simulink model "PID"  (R2025b)
settings: Solver=FixedStepAuto  StartTime=0.0  StopTime=10.0  FixedStep=0.01  RelTol=1e-3
undefined symbols (not defined in the file): b, c, g, I, kb, kt, l, M, m, r, Rm
libraries: vrlib x3, slpidlib x2
settings Model: Creator=jitendra  LastModifiedBy=joelalfaro
settings SolverCC: AlgebraicLoopSolver=TrustRegion
settings DataIOCC: ExternalInput=getinputstruct(op_trim1)  InitialState=getstatestruct(op_trim1)  ReturnWorkspaceOutputs=off
settings DebuggingCC: UnconnectedInputMsg=warning  UnconnectedOutputMsg=warning  UnconnectedLineMsg=warning  ArithmeticOperatorsInVariantConditions=warning
settings ModelReferenceCC: EnableRefExpFcnMdlSchedulingChecks=on
settings SFSimCC: SimUseLocalCustomCode=off  CustomCodeUndefinedFunction=UseInterfaceOnly
settings RTWCC: RTWUseLocalCustomCode=off  GPUComputeCapability=3.5

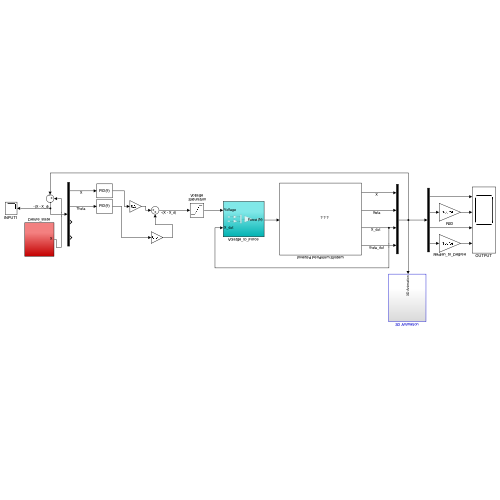
[thumbnail: Simulink's stored preview of the top-level diagram]
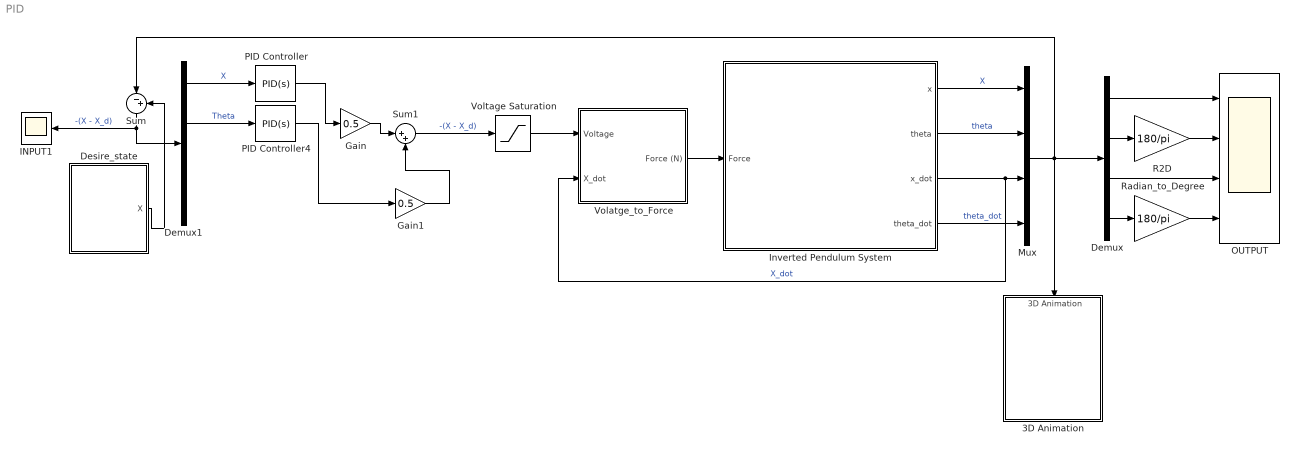
== system PID ==
  3D Animation : Subsystem
      settings: PortSchema="{\"entries\":[{\"content\":{\"sides\":[{\"content\":{},\"type\":\"ConnectorPlacement.EquallySpacedRectSide\",\"uuid\":\"e4203b7e-781e-4354-bf67-6c487e3884b6\"},{\"content\":{\"side\":\"RIGHT\"},\"type\":\"ConnectorPlacement.EquallySpacedRectSide\",\"uuid\":\"7bd3bb4e-855c-4795-9350-7e2ed6adbf10\"},{\"content\":{\"connectorIds\":[\"In1\"],\"side\":\"TOP\"},\"type\":\"ConnectorPlacement.EquallySpacedRectSide\",\"uuid\":\"c2ae83d0-35fa-4ceb-879c-e55f231126ee\"}]},\"type\":\"ConnectorPlacement.EquallySpacedConnector\",\"uuid\":\"fb632b4d-2504-45df-9ed9-db3d660227bd\"}],\"packageUris\":[\"http://schema.mathworks.com/mf0/Connector/R2020b\"],\"version\":\"1.0\"}"
  Demux : Demux
  Demux1 : Demux
  Desire_state : Subsystem
  Gain : Gain  Gain=0.5
  Gain1 : Gain  Gain=0.5
  INPUT1 : Scope
      settings: ActiveDisplayYMinimum=-15  ActiveDisplayYMaximum=15
  Inverted Pendulum System : Subsystem
      mask Display: image('ip_model.png');
  Mux : Mux
  OUTPUT : Scope  NumInputPorts=4
      settings: ActiveDisplayString=4  ActiveDisplayYMinimum=-139.60429875287392  ActiveDisplayYMaximum=335.60525389864625  YLabel=\theta dot (deg/sec)
  PID Controller : slpidlib/PID Controller  Controller=PID  Form=Parallel  TimeDomain=Continuous-time  UseExternalTs=off  SampleTime=-1  IntegratorMethod=Forward Euler  FilterMethod=Forward Euler  ControllerParametersSource=internal  P=-58.450  I=-25.45  UseKiTs=off  D=-5.57  UseExternalDerivativeSource=off  N=100  UseFilter=on  TunerSelectOption=Transfer Function Based (PID Tuner App)  InitialConditionSource=internal  InitialConditionForIntegrator=0  InitialConditionForFilter=0  DifferentiatorICPrevScaledInput=0  ExternalReset=none  TrackingMode=off  Kt=1  LimitOutput=off  SatLimitsSource=internal  UpperSaturationLimit=inf  LowerSaturationLimit=-inf  LinearizeAsGain=on  AntiWindupMode=none  Kb=1  LimitIntegrator=off  UpperIntegratorSaturationLimit=inf  LowerIntegratorSaturationLimit=-inf  POutMin=[]  POutMax=[]  IOutMin=[]  IOutMax=[]  DOutMin=[]  DOutMax=[]  NOutMin=[]  NOutMax=[]  SumOutMin=[]  SumOutMax=[]  SaturationOutMin=[]  SaturationOutMax=[]  PParamMin=[]  PParamMax=[]  IParamMin=[]  IParamMax=[]  DParamMin=[]  DParamMax=[]  NParamMin=[]  NParamMax=[]  KbParamMin=[]  KbParamMax=[]  KtParamMin=[]  KtParamMax=[]  KbOutMin=[]  KbOutMax=[]  KtOutMin=[]  KtOutMax=[]  IntegratorOutMin=[]  IntegratorOutMax=[]  FilterOutMin=[]  FilterOutMax=[]  SumI1OutMin=[]  SumI1OutMax=[]  SumI2OutMin=[]  SumI2OutMax=[]  SumI3OutMin=[]  SumI3OutMax=[]  SumI4OutMin=[]  SumI4OutMax=[]  SumDOutMin=[]  SumDOutMax=[]  DifferentiatorOutMin=[]  DifferentiatorOutMax=[]  FilterDiffOutCoefMin=[]  FilterDiffOutCoefMax=[]  ReciprocalOutMin=[]  ReciprocalOutMax=[]  SumDenOutMin=[]  SumDenOutMax=[]  SumNumOutMin=[]  SumNumOutMax=[]  DivideOutMin=[]  DivideOutMax=[]  UdiffTsProdOutMin=[]  UdiffTsProdOutMax=[]  NTsProdOutMin=[]  NTsProdOutMax=[]  UintegralTsProdOutMin=[]  UintegralTsProdOutMax=[]  UngainTsProdOutMin=[]  UngainTsProdOutMax=[]  ClampingZeroOutDataTypeStr=Inherit: Inherit via back propagation  ClampingZeroOutMin=[]  ClampingZeroOutMax=[]  FilterDenConstantOutDataTypeStr=Inherit: Inherit via back propagation  FilterDenConstantOutMin=[]  FilterDenConstantOutMax=[]  PCopyOutDataTypeStr=Inherit: Inherit via back propagation  PCopyOutMin=[]  PCopyOutMax=[]  NCopyOutDataTypeStr=Inherit: Inherit via back propagation  NCopyOutMin=[]  NCopyOutMax=[]  IntegratorContinuousStateAttributes=''  IntegratorStateMustResolveToSignalObject=off  IntegratorRTWStateStorageClass=Auto  FilterContinuousStateAttributes=''  FilterStateMustResolveToSignalObject=off  FilterRTWStateStorageClass=Auto  ParallelPVariant=InternalParameters  IdealPVariant=Disabled  IVariant=InternalParameters  DVariant=InternalParameters  IntegratorVariant=Continuous  SatVariant=Disabled  AWVariant=Passthrough  PCopyVariant=Disabled  TRVariant=Disabled  FdbkBlocksVariant=Forward  IdealPFdbkVariant=Disabled  SatFdbkVariant=Disabled  DerivativeFilterVariant=ContFilter  NVariant=InternalParameters  NCopyVariant=Disabled  FilterICVariant=InternalICsFilter  IntegratorICVariant=InternalICs  ExternalResetVariant=Disabled  TRSumVariant=Passthrough  SumFdbkVariant=Disabled  SumVariant=Sum_PID  TsampFilterVariant=InternalTs  TsampNgainVariant=Passthrough  TsampIntegralVariant=Disabled_SignalSpec  ExternalSaturationOutDataTypeStr=Inherit: Same as second input  DerivativeSourceVariant=ErrorSignal  PreIntVariant=InternalPreInt
  PID Controller4 : slpidlib/PID Controller  Controller=PID  Form=Parallel  TimeDomain=Continuous-time  UseExternalTs=off  SampleTime=-1  IntegratorMethod=Forward Euler  FilterMethod=Forward Euler  ControllerParametersSource=internal  P=120.5493  I=775.1235  UseKiTs=off  D=5.2021  UseExternalDerivativeSource=off  N=100  UseFilter=on  TunerSelectOption=Transfer Function Based (PID Tuner App)  InitialConditionSource=internal  InitialConditionForIntegrator=0  InitialConditionForFilter=0  DifferentiatorICPrevScaledInput=0  ExternalReset=none  TrackingMode=off  Kt=1  LimitOutput=off  SatLimitsSource=internal  UpperSaturationLimit=inf  LowerSaturationLimit=-inf  LinearizeAsGain=on  AntiWindupMode=none  Kb=1  LimitIntegrator=off  UpperIntegratorSaturationLimit=inf  LowerIntegratorSaturationLimit=-inf  POutMin=[]  POutMax=[]  IOutMin=[]  IOutMax=[]  DOutMin=[]  DOutMax=[]  NOutMin=[]  NOutMax=[]  SumOutMin=[]  SumOutMax=[]  SaturationOutMin=[]  SaturationOutMax=[]  PParamMin=[]  PParamMax=[]  IParamMin=[]  IParamMax=[]  DParamMin=[]  DParamMax=[]  NParamMin=[]  NParamMax=[]  KbParamMin=[]  KbParamMax=[]  KtParamMin=[]  KtParamMax=[]  KbOutMin=[]  KbOutMax=[]  KtOutMin=[]  KtOutMax=[]  IntegratorOutMin=[]  IntegratorOutMax=[]  FilterOutMin=[]  FilterOutMax=[]  SumI1OutMin=[]  SumI1OutMax=[]  SumI2OutMin=[]  SumI2OutMax=[]  SumI3OutMin=[]  SumI3OutMax=[]  SumI4OutMin=[]  SumI4OutMax=[]  SumDOutMin=[]  SumDOutMax=[]  DifferentiatorOutMin=[]  DifferentiatorOutMax=[]  FilterDiffOutCoefMin=[]  FilterDiffOutCoefMax=[]  ReciprocalOutMin=[]  ReciprocalOutMax=[]  SumDenOutMin=[]  SumDenOutMax=[]  SumNumOutMin=[]  SumNumOutMax=[]  DivideOutMin=[]  DivideOutMax=[]  UdiffTsProdOutMin=[]  UdiffTsProdOutMax=[]  NTsProdOutMin=[]  NTsProdOutMax=[]  UintegralTsProdOutMin=[]  UintegralTsProdOutMax=[]  UngainTsProdOutMin=[]  UngainTsProdOutMax=[]  ClampingZeroOutDataTypeStr=Inherit: Inherit via back propagation  ClampingZeroOutMin=[]  ClampingZeroOutMax=[]  FilterDenConstantOutDataTypeStr=Inherit: Inherit via back propagation  FilterDenConstantOutMin=[]  FilterDenConstantOutMax=[]  PCopyOutDataTypeStr=Inherit: Inherit via back propagation  PCopyOutMin=[]  PCopyOutMax=[]  NCopyOutDataTypeStr=Inherit: Inherit via back propagation  NCopyOutMin=[]  NCopyOutMax=[]  IntegratorContinuousStateAttributes=''  IntegratorStateMustResolveToSignalObject=off  IntegratorRTWStateStorageClass=Auto  FilterContinuousStateAttributes=''  FilterStateMustResolveToSignalObject=off  FilterRTWStateStorageClass=Auto  ParallelPVariant=InternalParameters  IdealPVariant=Disabled  IVariant=InternalParameters  DVariant=InternalParameters  IntegratorVariant=Continuous  SatVariant=Disabled  AWVariant=Passthrough  PCopyVariant=Disabled  TRVariant=Disabled  FdbkBlocksVariant=Forward  IdealPFdbkVariant=Disabled  SatFdbkVariant=Disabled  DerivativeFilterVariant=ContFilter  NVariant=InternalParameters  NCopyVariant=Disabled  FilterICVariant=InternalICsFilter  IntegratorICVariant=InternalICs  ExternalResetVariant=Disabled  TRSumVariant=Passthrough  SumFdbkVariant=Disabled  SumVariant=Sum_PID  TsampFilterVariant=InternalTs  TsampNgainVariant=Passthrough  TsampIntegralVariant=Disabled_SignalSpec  ExternalSaturationOutDataTypeStr=Inherit: Same as second input  DerivativeSourceVariant=ErrorSignal  PreIntVariant=InternalPreInt
  R2D : Gain  Gain=180/pi
  Radian_to_Degree : Gain  Gain=180/pi
  Sum : Sum  Inputs=|-+
  Sum1 : Sum  Inputs=|++
  Volatge_to_Force : Subsystem
  Voltage Saturation : Saturate  UpperLimit=12  LowerLimit=-12
  wires:
  Inverted Pendulum System/3(x_dot) -> Volatge_to_Force/2(X_dot), Mux/3  "X_dot"
  Inverted Pendulum System/2(theta) -> Mux/2  "theta"
  Inverted Pendulum System/1(x) -> Mux/1  "X"
  Inverted Pendulum System/4(theta_dot) -> Mux/4  "theta_dot"
  Mux/1 -> Sum/1, Demux/1, 3D Animation/1(3D Animation)
  Volatge_to_Force/1(Force (N)) -> Inverted Pendulum System/1(Force)
  Desire_state/1(X) -> Sum/2
  Voltage Saturation/1 -> Volatge_to_Force/1(Voltage)
  Demux/2 -> R2D/1
  Demux/1 -> OUTPUT/1
  Demux/3 -> OUTPUT/3
  Demux/4 -> Radian_to_Degree/1
  R2D/1 -> OUTPUT/2
  Radian_to_Degree/1 -> OUTPUT/4
  Sum/1 -> Demux1/1, INPUT1/1  "-(X - X_d)"
  Demux1/1 -> PID Controller/1  "X"
  Demux1/2 -> PID Controller4/1  "Theta"
  Sum1/1 -> Voltage Saturation/1  "-(X - X_d)"
  PID Controller4/1 -> Gain1/1
  PID Controller/1 -> Gain/1
  Gain/1 -> Sum1/1
  Gain1/1 -> Sum1/2

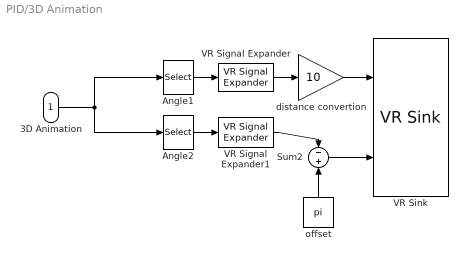
== system PID/3D Animation ==
  3D Animation : Inport
  Angle1 : Selector  InputPortWidth=4  IndexOptions=Index vector (dialog)  Indices=[1]  OutputSizes=1
  Angle2 : Selector  InputPortWidth=4  IndexOptions=Index vector (dialog)  Indices=[2]  OutputSizes=1
  Sum2 : Sum  Inputs=-|+
  VR Signal Expander : vrlib/VR Signal Expander  outwidth=3  outidx=[1]
  VR Signal Expander1 : vrlib/VR Signal Expander  outwidth=4  outidx=[4]
  VR Sink : vrlib/VR Sink  InstantiateOnLoad=on  SampleTime=0.02  ViewEnable=on  RemoteChange=off  RemoteView=off  FieldsWritten=cart.translation.3.1.1.double#joint.rotation.4.1.1.double  WorldFileName=Inverted_pendulum12.wrl  AutoView=off  VideoDimensions=[]  AllowVariableSize=off  FigureProperties="{'Position', 'Name', 'Viewpoint', 'CameraBound', 'CameraDirection', 'CameraPosition', 'CameraUpVector', 'ZoomFactor', 'Antialiasing', 'Headlight', 'Lighting', 'Sound', 'StatusBar', 'Stereo3D', 'Stereo3DCameraOffset', 'Stereo3DHIT', 'ToolBar', 'Textures', 'Transparency', 'Triad', 'Wireframe', 'NavZones', 'NavMode', 'NavSpeed', 'CaptureFileFormat', 'CaptureFileName', 'Record2DCompressMethod', 'Record2DCompressQuality', 'Record2D', 'Record2DFileName', 'Record2DFPS'; [5.0000000000000000e+00   9.2000000000000000e+01   5.7600000000000000e+02   3.8000000000000000e+02], '', '\"\"', 'on', [0.0000000000000000e+00   0.0000000000000000e+00  -1.0000000000000000e+00], [0.0000000000000000e+00   0.0000000000000000e+00   0.0000000000000000e+00], [0.0000000000000000e+00   1.0000000000000000e+00   0.0000000000000000e+00], [1.0000000000000000e+00], 'on', 'on', 'on', 'off', 'on', 'off', [1.0000000000000001e-01], [0.0000000000000000e+00], 'on', 'on', 'on', 'none', 'off', 'off', 'examine', 'normal', 'tif', '%f_anim_%n.tif', 'auto', [7.5000000000000000e+01], 'off', '%f_anim_%n.avi', 'auto'}"
  distance convertion : Gain  Gain=10
  offset : Constant  Value=pi
  wires:
  VR Signal Expander/1 -> distance convertion/1
  3D Animation/1 -> Angle2/1, Angle1/1
  Angle1/1 -> VR Signal Expander/1
  Angle2/1 -> VR Signal Expander1/1
  offset/1 -> Sum2/2
  Sum2/1 -> VR Sink/2
  VR Signal Expander1/1 -> Sum2/1
  distance convertion/1 -> VR Sink/1

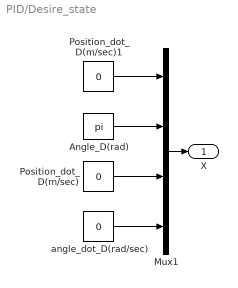
== system PID/Desire_state ==
  Angle_D(rad) : Constant  Value=pi
  Mux1 : Mux
  Position_dot_D(m/sec) : Constant  Value=0
  Position_dot_D(m/sec)1 : Constant  Value=0
  angle_dot_D(rad/sec) : Constant  Value=0
  X : Outport  VectorParamsAs1DForOutWhenUnconnected=off
  wires:
  Mux1/1 -> X/1
  Position_dot_D(m/sec)/1 -> Mux1/3
  angle_dot_D(rad/sec)/1 -> Mux1/4
  Angle_D(rad)/1 -> Mux1/2
  Position_dot_D(m/sec)1/1 -> Mux1/1

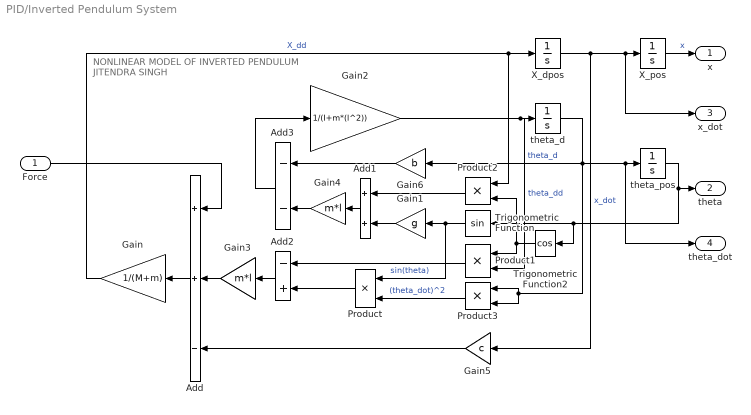
== system PID/Inverted Pendulum System ==
  note: NONLINEAR MODEL OF
      | INVERTED PENDULUM
      | JITENDRA SINGH
  Force : Inport
  Add : Sum  Inputs=++-
  Add1 : Sum
  Add2 : Sum  Inputs=-+
  Add3 : Sum  Inputs=--
  Gain : Gain  Gain=1/(M+m)
  Gain1 : Gain  Gain=g
  Gain2 : Gain  Gain=1/(I+m*(l^2))
  Gain3 : Gain  Gain=m*l
  Gain4 : Gain  Gain=m*l
  Gain5 : Gain  Gain=c
  Gain6 : Gain  Gain=b
  Product{,1..3} (4 alike) : Product
  Trigonometric Function : Trigonometry
  Trigonometric Function2 : Trigonometry  Operator=cos
  X_dpos : Integrator
  X_pos : Integrator  InitialCondition=0.2
  theta_d : Integrator
  theta_pos : Integrator  InitialCondition=160*(pi/180)
  x : Outport  VectorParamsAs1DForOutWhenUnconnected=off
  theta : Outport  Port=2  VectorParamsAs1DForOutWhenUnconnected=off
  x_dot : Outport  Port=3  VectorParamsAs1DForOutWhenUnconnected=off
  theta_dot : Outport  Port=4  VectorParamsAs1DForOutWhenUnconnected=off
  wires:
  Gain5/1 -> Add/3
  Add2/1 -> Gain3/1
  Add3/1 -> Gain2/1
  Trigonometric Function2/1 -> Product2/2, Product1/1
  Trigonometric Function/1 -> Product/1, Gain1/1  "sin(theta)"
  Gain3/1 -> Add/2
  theta_d/1 -> Product3/2, Product3/1, Gain6/1, theta_dot/1, theta_pos/1  "theta_d"
  Product2/1 -> Add1/1
  Product/1 -> Add2/2
  Gain4/1 -> Add3/2
  Product3/1 -> Product/2  "(theta_dot)^2"
  X_pos/1 -> x/1  "x"
  Product1/1 -> Add2/1
  Gain/1 -> X_dpos/1, Product2/1  "X_dd"
  Add/1 -> Gain/1
  Gain2/1 -> Product1/2, theta_d/1  "theta_dd"
  Gain6/1 -> Add3/1
  theta_pos/1 -> Trigonometric Function2/1, Trigonometric Function/1, theta/1
  Force/1 -> Add/1
  Gain1/1 -> Add1/2
  X_dpos/1 -> x_dot/1, X_pos/1, Gain5/1  "x_dot"
  Add1/1 -> Gain4/1

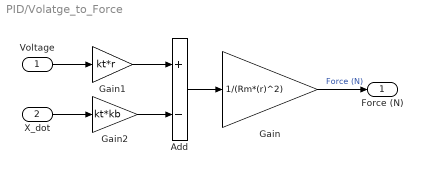
== system PID/Volatge_to_Force ==
  Voltage : Inport
  X_dot : Inport  Port=2
  Add : Sum  Inputs=+-
  Gain : Gain  Gain=1/(Rm*(r)^2)
  Gain1 : Gain  Gain=kt*r
  Gain2 : Gain  Gain=kt*kb
  Force (N) : Outport  VectorParamsAs1DForOutWhenUnconnected=off
  wires:
  Gain1/1 -> Add/1
  Gain2/1 -> Add/2
  Voltage/1 -> Gain1/1
  Gain/1 -> Force (N)/1  "Force (N)"
  X_dot/1 -> Gain2/1
  Add/1 -> Gain/1
